simulink model "FMT_G1_OrderedWorker"  (R2026b)
settings: Solver=FixedStepDiscrete  StopTime=2  FixedStep=0.0005
settings Model: Creator=26718  LastModifiedBy=26718

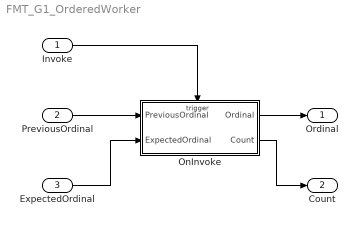
== system FMT_G1_OrderedWorker ==
  Invoke : Inport  OutputFunctionCall=on
  PreviousOrdinal : Inport  Port=2  OutDataTypeStr=uint64
  ExpectedOrdinal : Inport  Port=3  OutDataTypeStr=uint64
  OnInvoke : Subsystem
  Ordinal : Outport
  Count : Outport  Port=2
  wires:
  OnInvoke/2(Count) -> Count/1
  OnInvoke/1(Ordinal) -> Ordinal/1
  ExpectedOrdinal/1 -> OnInvoke/2(ExpectedOrdinal)
  PreviousOrdinal/1 -> OnInvoke/1(PreviousOrdinal)
  Invoke/1 -> OnInvoke/Trigger

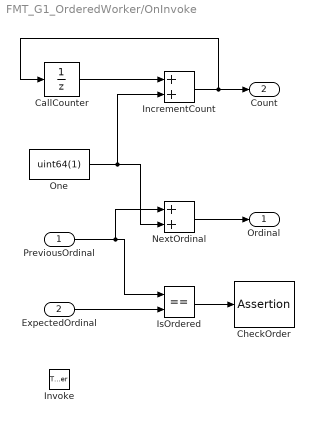
== system FMT_G1_OrderedWorker/OnInvoke ==
  PreviousOrdinal : Inport
  ExpectedOrdinal : Inport  Port=2
  Invoke : TriggerPort  TriggerType=function-call  VariantControl=(inherit)  PortDimensions=1
  CallCounter : UnitDelay  InitialCondition=uint64(0)  SampleTime=-1
  CheckOrder : Assertion
  IncrementCount : Sum  OutDataTypeStr=uint64
  IsOrdered : RelationalOperator  Operator===  OutDataTypeStr=boolean  RndMeth=Simplest  InputSameDT=off
  NextOrdinal : Sum  OutDataTypeStr=uint64
  One : Constant  Value=uint64(1)  OutDataTypeStr=uint64
  Ordinal : Outport
  Count : Outport  Port=2
  wires:
  IncrementCount/1 -> CallCounter/1, Count/1
  CallCounter/1 -> IncrementCount/1
  IsOrdered/1 -> CheckOrder/1
  ExpectedOrdinal/1 -> IsOrdered/2
  NextOrdinal/1 -> Ordinal/1
  One/1 -> NextOrdinal/2, IncrementCount/2
  PreviousOrdinal/1 -> IsOrdered/1, NextOrdinal/1
